simulink model "EI7_V2_R2024a"  (R2018b)
settings: Solver=ode23tb  StartTime=0.0  StopTime=0.5  MaxStep=5e-4  RelTol=1e-5  AbsTol=1e-6
values from neighbouring files (symbols this model uses):
  feder_M_lut = [-0.20, -0.022, -0.015,  0.000,  0.015,  0.022,  0.15,  0.50]    [init_parameters.m]
  feder_phi_lut = [-0.5,   0.0,    7.4,    7.5,    7.6,    90.0,   90.1,  91.0]    [init_parameters.m]
  J_ges = 7.2e-6    (= 7.2e-06)    [init_parameters.m]
  k_EMK = 0.030    (= 0.03)    [init_parameters.m]
  K_Gr = 1.0 / i_Getr    (= 0.05)    [init_parameters.m]
  k_Mot = 0.027    [init_parameters.m]
  phi_0_rad = phi_0_deg * pi / 180.0    (= 0.1308996939)    [init_parameters.m]
  reib_M_lut = [-M_R,  -M_R,  0.0,  M_R,  M_R]    [init_parameters.m]
  reib_w_lut = [-1000, -0.5,  0.0,  0.5,  1000]    [init_parameters.m]
  t_step = 0.05    [init_parameters.m]
  U_step_val = 6.0    (= 6)    [init_parameters.m]
settings Model: Creator=grund  LastModifiedBy=grund
settings DataIOCC: ReturnWorkspaceOutputs=on
settings DebuggingCC: UnconnectedInputMsg=none  UnconnectedOutputMsg=none  UnconnectedLineMsg=none
settings ModelReferenceCC: EnableRefExpFcnMdlSchedulingChecks=off
settings RTWCC: Description=Generic Real-Time Target
settings ConfigComp: CovBoundaryAbsTol=1.0e-5

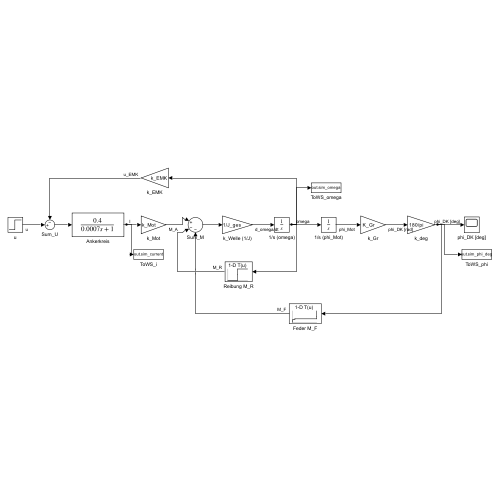
[thumbnail: Simulink's stored preview of the top-level diagram]
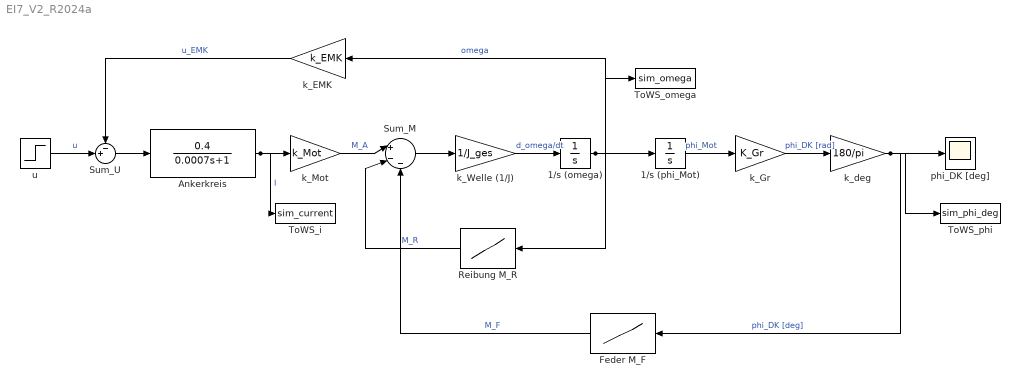
== system EI7_V2_R2024a ==
  1/s (omega) : Integrator
  1/s (phi_Mot) : Integrator  InitialCondition=phi_0_rad / K_Gr
  Ankerkreis : TransferFcn  Numerator=[0.4]  Denominator=[0.0007 1]
  Feder M_F : Lookup_n-D  NumberOfTableDimensions=1  BreakpointsForDimension1=feder_phi_lut  Table=feder_M_lut  InternalRulePriority=Speed  RndMeth=Simplest  InputSameDT=on
  Reibung M_R : Lookup_n-D  NumberOfTableDimensions=1  BreakpointsForDimension1=reib_w_lut  Table=reib_M_lut  InternalRulePriority=Speed  RndMeth=Simplest  InputSameDT=on
  Sum_M : Sum  Inputs=|+--
  Sum_U : Sum  Inputs=-+|
  ToWS_i : ToWorkspace  VariableName=sim_current  SaveFormat=Timeseries  SampleTime=-1
  ToWS_omega : ToWorkspace  VariableName=sim_omega  SaveFormat=Timeseries  SampleTime=-1
  ToWS_phi : ToWorkspace  VariableName=sim_phi_deg  SaveFormat=Timeseries  SampleTime=-1
  k_EMK : Gain  Gain=k_EMK
  k_Gr : Gain  Gain=K_Gr
  k_Mot : Gain  Gain=k_Mot
  k_Welle (1/J) : Gain  Gain=1/J_ges
  k_deg : Gain  Gain=180/pi
  phi_DK [deg] : Scope
  u : Step  Time=t_step  After=U_step_val  SampleTime=0
  wires:
  u/1 -> Sum_U/2  "u"
  Sum_U/1 -> Ankerkreis/1
  Ankerkreis/1 -> k_Mot/1, ToWS_i/1  "I"
  k_Mot/1 -> Sum_M/1  "M_A"
  Sum_M/1 -> k_Welle (1/J)/1
  k_Welle (1/J)/1 -> 1/s (omega)/1  "d_omega/dt"
  1/s (omega)/1 -> 1/s (phi_Mot)/1, k_EMK/1, Reibung M_R/1, ToWS_omega/1  "omega"
  1/s (phi_Mot)/1 -> k_Gr/1  "phi_Mot"
  k_Gr/1 -> k_deg/1  "phi_DK [rad]"
  k_deg/1 -> phi_DK [deg]/1, Feder M_F/1, ToWS_phi/1  "phi_DK [deg]"
  k_EMK/1 -> Sum_U/1  "u_EMK"
  Reibung M_R/1 -> Sum_M/2  "M_R"
  Feder M_F/1 -> Sum_M/3  "M_F"
